simulink model "chaine_hamming"  (R2023b)
settings: Solver=VariableStepAuto  StartTime=0.0  StopTime=200  RelTol=1e-3
values from neighbouring files (symbols this model uses):
  A = P.A    [P3_Q10_parametres_integration.m]    (also in P3_Q11_variance_integrateur.m; P3_Q12_TEB.m; P3_Q4_bruit_uniforme.m; P3_Q5_erreur_uniforme.m)
  L = P.L    [P3_Q10_parametres_integration.m]    (also in P3_Q11_variance_integrateur.m; P3_Q12_TEB.m; P3_Q13_integration.m; P3_parametres.m)
  P = parametres_perso('LABBE Emmy')    [P2_Q11_LZ78_convergence.m]    (also in P2_Q1_source_binaire_simulation.m; P2_Q7_extension_source.m; P3_Q10_parametres_integration.m; P3_Q11_variance_integrateur.m)
  Tb = 1;')    [LANCER_TP_COMPLET.m]    (also in P2_Q1_source_binaire_simulation.m = 1; P3_Q10_parametres_integration.m = 1; P3_Q11_variance_integrateur.m = 1; P3_Q12_TEB.m = 1)
  Te = Tb / L    [P3_Q10_parametres_integration.m]    (also in P3_Q11_variance_integrateur.m; P3_Q12_TEB.m; P3_parametres.m = Tb/L)
libraries: simulink x2, dspstat3 x1
settings Model: Creator=e2202522  LastModifiedBy=e2202522

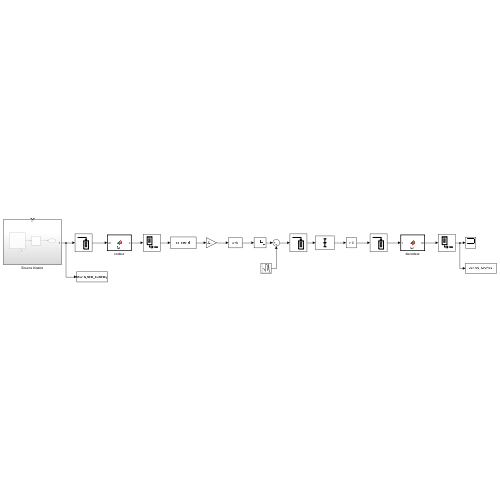
[thumbnail: Simulink's stored preview of the top-level diagram]
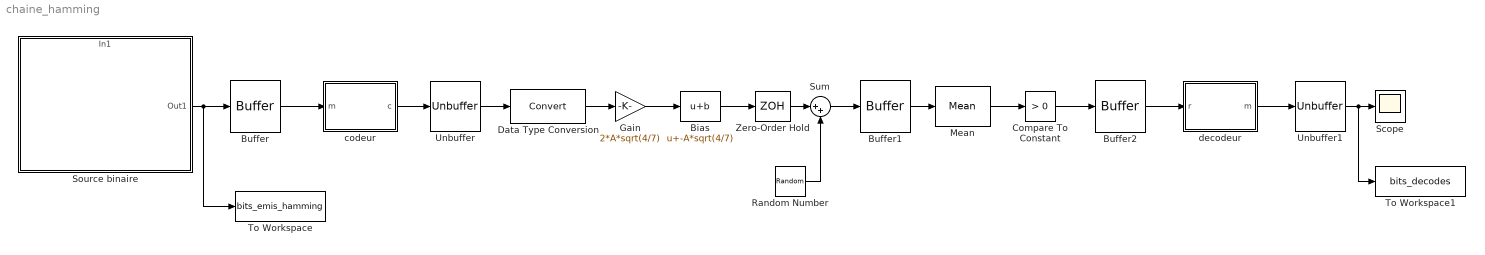
== system chaine_hamming ==
  Bias : Bias  Bias=-A*sqrt(4/7)  SaturateOnIntegerOverflow=off
  Buffer : Buffer  N=4  OutputFrames=off
  Buffer1 : Buffer  N=L  OutputFrames=off
  Buffer2 : Buffer  N=7  OutputFrames=off
  Compare To Constant : simulink/Logic and Bit Operations/Compare To Constant  relop=>  const=0  OutDataTypeStr=boolean
  Data Type Conversion : DataTypeConversion  SaturateOnIntegerOverflow=off  RndMeth=Floor
  Gain : Gain  Gain=2*A*sqrt(4/7)
  Mean : dspstat3/Mean  run=off  InputProcessing=Columns as channels (frame based)  reset_popup=None  directionMode=Each column  dimension=1  roiEnable=off  roiType=Rectangles  roiPortion=Entire ROI  roiOutput=Individual statistics for each ROI  roiFlag=off  roundingMode=Floor  overflowMode=off  outputDataTypeStr=Inherit: Same as accumulator  outputMin=[]  outputMax=[]  outputLastDataTypeStr=Inherit: Same as accumulator
  Random Number : RandomNumber  Variance=0  SampleTime=Te
  Scope : Scope
  Source binaire : Subsystem
      settings: PortSchema="{\"entries\":[{\"content\":{\"sides\":[{\"content\":{},\"type\":\"ConnectorPlacement.EquallySpacedRectSide\",\"uuid\":\"1d1b3a40-eee1-4311-a28c-a5c990f69d61\"},{\"content\":{\"connectorIds\":[\"Out1\"],\"side\":\"RIGHT\"},\"type\":\"ConnectorPlacement.EquallySpacedRectSide\",\"uuid\":\"9115f35c-513c-4ea1-a40d-1e1aebcfde17\"},{\"content\":{\"connectorIds\":[\"In1\"],\"side\":\"TOP\"},\"type\":\"ConnectorPlacement.EquallySpacedRectSide\",\"uuid\":\"a6426102-e6a6-474b-a4e7-9dc638e2ca24\"}]},\"type\":\"ConnectorPlacement.EquallySpacedConnector\",\"uuid\":\"766fcb99-2af9-4dfe-9edb-f04684085cad\"}],\"packageUris\":[\"http://schema.mathworks.com/mf0/Connector/R2020b\"],\"version\":\"1.0\"}"
  Sum : Sum  Inputs=|++
  To Workspace : ToWorkspace  VariableName=bits_emis_hamming  SampleTime=-1
  To Workspace1 : ToWorkspace  VariableName=bits_decodes  SampleTime=-1
  Unbuffer : Unbuffer
  Unbuffer1 : Unbuffer
  Zero-Order Hold : ZeroOrderHold  SampleTime=Te
  codeur : MATLAB Function  TreatAsAtomicUnit=on
  decodeur : MATLAB Function  TreatAsAtomicUnit=on
  wires:
  Source binaire/1(Out1) -> To Workspace/1, Buffer/1
  Buffer/1 -> codeur/1(m)
  codeur/1(c) -> Unbuffer/1
  Unbuffer/1 -> Data Type Conversion/1
  Data Type Conversion/1 -> Gain/1
  Gain/1 -> Bias/1
  Bias/1 -> Zero-Order Hold/1
  Zero-Order Hold/1 -> Sum/1
  Random Number/1 -> Sum/2
  Sum/1 -> Buffer1/1
  Buffer1/1 -> Mean/1
  Mean/1 -> Compare To Constant/1
  Compare To Constant/1 -> Buffer2/1
  Buffer2/1 -> decodeur/1(r)
  decodeur/1(m) -> Unbuffer1/1
  Unbuffer1/1 -> To Workspace1/1, Scope/1

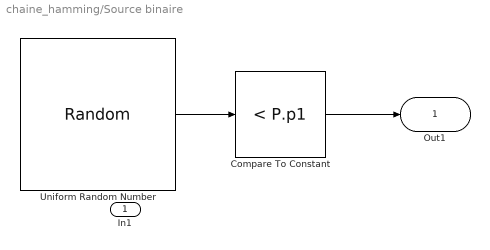
== system chaine_hamming/Source binaire ==
  In1 : Inport
  Compare To Constant : simulink/Logic and Bit Operations/Compare To Constant  relop=<  const=P.p1  OutDataTypeStr=boolean
  Uniform Random Number : UniformRandomNumber  Minimum=0  Seed=P.graine  SampleTime=Tb
  Out1 : Outport
  wires:
  Compare To Constant/1 -> Out1/1
  Uniform Random Number/1 -> Compare To Constant/1

== matlab function chaine_hamming/codeur ==
  data: m input; c output
function c = fcn(m)

P = [
    1 1 0;
    0 1 1;
    1 1 1;
    1 0 1
];

G = [eye(4) P];

% Message sous forme de ligne
m_ligne = double(m(:).');

% Codage Hamming
temp = mod(m_ligne * G, 2);

% Sortie toujours en colonne 7x1
c = temp(:);

end

== matlab function chaine_hamming/decodeur ==
  data: r input; m output
function m = fcn(r)

P = [
    1 1 0;
    0 1 1;
    1 1 1;
    1 0 1
];

H = [P' eye(3)];

% Passage en ligne
r_ligne = double(r(:).');

% Calcul du syndrome
syndrome = mod(r_ligne * H', 2);

% Copie du mot recu
r_corrige = r_ligne;

% Recherche de la position de l'erreur
for i = 1:7

    if isequal(syndrome, H(:,i)')
        r_corrige(i) = 1 - r_corrige(i);
        break;
    end

end

% Le code est systematique :
% les 4 premiers bits correspondent au message
temp = r_corrige(1:4);

% Sortie en colonne 4x1
m = temp(:);

end
